simulink library "casper_library_delays"  (Simulink 7.2)
settings: Solver=ode45  SolverMode=SingleTasking  StartTime=0.0  StopTime=10.0  RelTol=1e-3
libraries: xbsIndex_r4 x378, casper_library_misc x18, casper_library_delays x16, xbsReplacements_r4 x5, casper_library_multipliers x4, casper_library_downconverter x2
(part 5 of 5)

== system casper_library_delays/finedelay_fstop_prog_cordic/CORDIC_SINCOS2/CORDIC Fine Angle PE/CORDIC PE8 ==
  note: X = x + y if z < 0, otherwise
      |    = x - y
      | Y = y - x if z < 0, otherwise
      |    = y + x
      | Z = z + atan(1/2^i) if z < 0, otherwise
      |    = z - atan(1/2^i)
  x : Inport
  y : Inport  Port=2
  z : Inport  Port=3
  AddSub : xbsIndex_r4/AddSub  mode=Addition or Subtraction  use_carryin=off  use_carryout=off  en=off  latency=pipeline  precision=User Defined  arith_type="Signed  (2's comp)"  n_bits=pe_nbits  bin_pt=pe_binpt  quantization=Truncate  overflow=Wrap  dbl_ovrd=off  use_behavioral_HDL=on  hw_selection=Fabric  pipelined=off  use_rpm=off  block_type=addsub
      settings: xl_area=[8 16 0 16 0 0 0]  block_version=VER_STRING_GOES_HERE
  AddSub1 : xbsIndex_r4/AddSub  mode=Addition or Subtraction  use_carryin=off  use_carryout=off  en=off  latency=pipeline  precision=User Defined  arith_type="Signed  (2's comp)"  n_bits=pe_nbits  bin_pt=pe_binpt  quantization=Truncate  overflow=Wrap  dbl_ovrd=off  use_behavioral_HDL=on  hw_selection=Fabric  pipelined=off  use_rpm=off  block_type=addsub
      settings: xl_area=[8 16 0 16 0 0 0]  block_version=VER_STRING_GOES_HERE
  AddSub2 : xbsIndex_r4/AddSub  mode=Addition or Subtraction  use_carryin=off  use_carryout=off  en=off  latency=pipeline  precision=User Defined  arith_type="Signed  (2's comp)"  n_bits=pe_nbits  bin_pt=pe_binpt  quantization=Truncate  overflow=Wrap  dbl_ovrd=off  use_behavioral_HDL=on  hw_selection=Fabric  pipelined=off  use_rpm=off  block_type=addsub
      settings: xl_area=[8 16 0 16 0 0 0]  block_version=VER_STRING_GOES_HERE
  Constant : xbsIndex_r4/Constant  const=epsilon_k  gui_display_data_type=Fixed-point  arith_type=Signed (2's comp)  n_bits=pe_nbits  bin_pt=pe_binpt  preci_type=Single  exp_width=8  frac_width=24  explicit_period=off  period=1  equ=P=C  opselect=C  inp2=PCIN>>17  opr=+  inp1=P  carry=CIN  dbl_ovrd=off  block_type=constant
      settings: block_version=VER_STRING_GOES_HERE
  Inverter : xbsIndex_r4/Inverter  en=off  latency=0  dbl_ovrd=off  block_type=inv
      settings: xl_area=[1 0 0 1 0 0 0]  block_version=VER_STRING_GOES_HERE
  Shift : xbsIndex_r4/Shift  shift_dir=Right  shift_bits=ii  en=off  latency=0  precision=User Defined  arith_type="Signed  (2's comp)"  n_bits=pe_nbits  bin_pt=pe_binpt  quantization=Truncate  overflow=Wrap  dbl_ovrd=off  block_type=shift
      settings: xl_area=[0 0 0 0 0 0 0]  block_version=VER_STRING_GOES_HERE
  Shift1 : xbsIndex_r4/Shift  shift_dir=Right  shift_bits=ii  en=off  latency=0  precision=User Defined  arith_type="Signed  (2's comp)"  n_bits=pe_nbits  bin_pt=pe_binpt  quantization=Truncate  overflow=Wrap  dbl_ovrd=off  block_type=shift
      settings: xl_area=[0 0 0 0 0 0 0]  block_version=VER_STRING_GOES_HERE
  Slice : xbsIndex_r4/Slice  nbits=1  boolean_output=on  mode=Upper Bit Location + Width  bit1=0  base1=MSB of Input  bit0=0  base0=LSB of Input  dbl_ovrd=off  block_type=slice
      settings: infoedit="Extracts a given range of bits from each input sample and presents it at the output.  The output type is ordinarily unsigned with binary point at zero, but can be Boolean when the slice is one bit wide.<P><P>Hardware notes: In hardware this block costs nothing."  block_version=VER_STRING_GOES_HERE
  X : Outport
  Y : Outport  Port=2
  Z : Outport  Port=3
  wires:
  Inverter/1 -> AddSub/3, AddSub2/3
  Slice/1 -> AddSub1/3, Inverter/1
  Shift1/1 -> AddSub/2
  Shift/1 -> AddSub1/2
  Constant/1 -> AddSub2/2
  AddSub2/1 -> Z/1
  AddSub1/1 -> Y/1
  z/1 -> Slice/1, AddSub2/1
  AddSub/1 -> X/1
  y/1 -> Shift1/1, AddSub1/1
  x/1 -> Shift/1, AddSub/1

== system casper_library_delays/finedelay_fstop_prog_cordic/CORDIC_SINCOS2/CORDIC Fine Angle PE/CORDIC PE9 ==
  note: X = x + y if z < 0, otherwise
      |    = x - y
      | Y = y - x if z < 0, otherwise
      |    = y + x
      | Z = z + atan(1/2^i) if z < 0, otherwise
      |    = z - atan(1/2^i)
  x : Inport
  y : Inport  Port=2
  z : Inport  Port=3
  AddSub : xbsIndex_r4/AddSub  mode=Addition or Subtraction  use_carryin=off  use_carryout=off  en=off  latency=pipeline  precision=User Defined  arith_type="Signed  (2's comp)"  n_bits=pe_nbits  bin_pt=pe_binpt  quantization=Truncate  overflow=Wrap  dbl_ovrd=off  use_behavioral_HDL=on  hw_selection=Fabric  pipelined=off  use_rpm=off  block_type=addsub
      settings: xl_area=[8 16 0 16 0 0 0]  block_version=VER_STRING_GOES_HERE
  AddSub1 : xbsIndex_r4/AddSub  mode=Addition or Subtraction  use_carryin=off  use_carryout=off  en=off  latency=pipeline  precision=User Defined  arith_type="Signed  (2's comp)"  n_bits=pe_nbits  bin_pt=pe_binpt  quantization=Truncate  overflow=Wrap  dbl_ovrd=off  use_behavioral_HDL=on  hw_selection=Fabric  pipelined=off  use_rpm=off  block_type=addsub
      settings: xl_area=[8 16 0 16 0 0 0]  block_version=VER_STRING_GOES_HERE
  AddSub2 : xbsIndex_r4/AddSub  mode=Addition or Subtraction  use_carryin=off  use_carryout=off  en=off  latency=pipeline  precision=User Defined  arith_type="Signed  (2's comp)"  n_bits=pe_nbits  bin_pt=pe_binpt  quantization=Truncate  overflow=Wrap  dbl_ovrd=off  use_behavioral_HDL=on  hw_selection=Fabric  pipelined=off  use_rpm=off  block_type=addsub
      settings: xl_area=[8 16 0 16 0 0 0]  block_version=VER_STRING_GOES_HERE
  Constant : xbsIndex_r4/Constant  const=epsilon_k  gui_display_data_type=Fixed-point  arith_type=Signed (2's comp)  n_bits=pe_nbits  bin_pt=pe_binpt  preci_type=Single  exp_width=8  frac_width=24  explicit_period=off  period=1  equ=P=C  opselect=C  inp2=PCIN>>17  opr=+  inp1=P  carry=CIN  dbl_ovrd=off  block_type=constant
      settings: block_version=VER_STRING_GOES_HERE
  Inverter : xbsIndex_r4/Inverter  en=off  latency=0  dbl_ovrd=off  block_type=inv
      settings: xl_area=[1 0 0 1 0 0 0]  block_version=VER_STRING_GOES_HERE
  Shift : xbsIndex_r4/Shift  shift_dir=Right  shift_bits=ii  en=off  latency=0  precision=User Defined  arith_type="Signed  (2's comp)"  n_bits=pe_nbits  bin_pt=pe_binpt  quantization=Truncate  overflow=Wrap  dbl_ovrd=off  block_type=shift
      settings: xl_area=[0 0 0 0 0 0 0]  block_version=VER_STRING_GOES_HERE
  Shift1 : xbsIndex_r4/Shift  shift_dir=Right  shift_bits=ii  en=off  latency=0  precision=User Defined  arith_type="Signed  (2's comp)"  n_bits=pe_nbits  bin_pt=pe_binpt  quantization=Truncate  overflow=Wrap  dbl_ovrd=off  block_type=shift
      settings: xl_area=[0 0 0 0 0 0 0]  block_version=VER_STRING_GOES_HERE
  Slice : xbsIndex_r4/Slice  nbits=1  boolean_output=on  mode=Upper Bit Location + Width  bit1=0  base1=MSB of Input  bit0=0  base0=LSB of Input  dbl_ovrd=off  block_type=slice
      settings: infoedit="Extracts a given range of bits from each input sample and presents it at the output.  The output type is ordinarily unsigned with binary point at zero, but can be Boolean when the slice is one bit wide.<P><P>Hardware notes: In hardware this block costs nothing."  block_version=VER_STRING_GOES_HERE
  X : Outport
  Y : Outport  Port=2
  Z : Outport  Port=3
  wires:
  Inverter/1 -> AddSub/3, AddSub2/3
  Slice/1 -> AddSub1/3, Inverter/1
  Shift1/1 -> AddSub/2
  Shift/1 -> AddSub1/2
  Constant/1 -> AddSub2/2
  AddSub2/1 -> Z/1
  AddSub1/1 -> Y/1
  z/1 -> Slice/1, AddSub2/1
  AddSub/1 -> X/1
  y/1 -> Shift1/1, AddSub1/1
  x/1 -> Shift/1, AddSub/1
